simulink model "deliverable_1_simulink"  (R2026a)
settings: Solver=ode4  StopTime=20  FixedStep=0.01
settings Model: Creator=20253802  LastModifiedBy=20253802

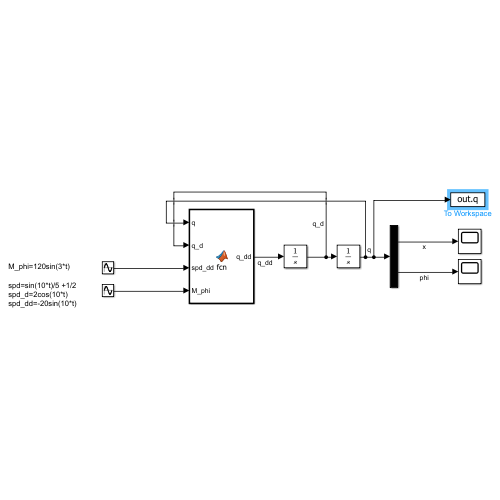
[thumbnail: Simulink's stored preview of the top-level diagram]
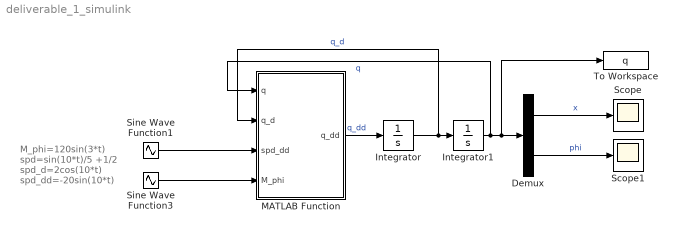
== system deliverable_1_simulink ==
  note: M_phi=120sin(3*t)
      |
      | spd=sin(10*t)/5 +1/2
      | spd_d=2cos(10*t)
      | spd_dd=-20sin(10*t)
  Demux : Demux  Outputs=2
  Integrator : Integrator  InitialCondition=[0 ; 0]
  Integrator1 : Integrator  InitialCondition=[0.1; -pi/4]
  MATLAB Function : MATLAB Function  TreatAsAtomicUnit=on
  Scope : Scope
      settings: ActiveDisplayYMinimum=0.2439492742252623  ActiveDisplayYMaximum=0.82436014260747192
  Scope1 : Scope
      settings: ActiveDisplayYMinimum=-3.2356158180174166  ActiveDisplayYMaximum=0.652208178898841
  Sine Wave Function1 : Sin  Amplitude=-20  Frequency=10  SampleTime=0
  Sine Wave Function3 : Sin  Amplitude=120  Frequency=3  SampleTime=0
  To Workspace : ToWorkspace  VariableName=q  SaveFormat=Timeseries  SampleTime=-1
  wires:
  MATLAB Function/1(q_dd) -> Integrator/1  "q_dd"
  Integrator/1 -> MATLAB Function/2(q_d), Integrator1/1  "q_d"
  Integrator1/1 -> To Workspace/1, Demux/1, MATLAB Function/1(q)  "q"
  Sine Wave Function1/1 -> MATLAB Function/3(spd_dd)
  Sine Wave Function3/1 -> MATLAB Function/4(M_phi)
  Demux/1 -> Scope/1  "x"
  Demux/2 -> Scope1/1  "phi"

== matlab function deliverable_1_simulink/MATLAB Function ==
  data: q input; q_dd output; q_d input; spd_dd input; M_phi input
function q_dd = fcn(q,q_d,spd_dd,M_phi)
%% System Parameters

% Gravitational acceleration
g = 9.81;               % [m/s^2]

% Geometry
L23 = 0.05;             % Distance between points 2 and 3 [m]

% Masses
mc = 2.0;               % Mass of carriage [kg]
mh = 0.7;               % Mass of milling head [kg]

% Inertia
Jh2 = 1.2;              % Rotational inertia of milling head about point 2 [kg*m^2]

% PD controller (x-direction)
kPD = 380;              % Proportional gain [N/m]
xPD_ref = 0.5;          % Reference position [m]
dPD = 10;               % Derivative gain [N*s/m]

% Translational spring-damper (between points 1 and 2)
dx = 0.5;               % Damping coefficient [N*s/m]

% Rotational spring-damper
kphi = 100;             % Rotational stiffness [N*m/rad]

% For problems except D5.f and D6
dphi = 2;               % Rotational damping [N*m*s/rad]

% Reference angles
phi_ref = -0.5*pi;      % Reference angle of band brake [rad]
phi_h3 = (2/3)*pi;      % Relative angle of milling head [rad]



%Generalised coordinates

x     = q(1);
phi   = q(2);
x_d   = q_d(1);
phi_d = q_d(2);
phi3  = phi-phi_h3;

%Calculate M and F

M = [mc+mh,              -mh*L23*sin(phi3);
    -mh*L23*sin(phi3),   Jh2];

F = [
    mh*L23*cos(phi3)*phi_d^2 - kPD*(x - xPD_ref) - (dx + dPD)*x_d ;

    M_phi - mh*L23*cos(phi3)*spd_dd - mh*g*L23*cos(phi3) - kphi*(phi - phi_ref) - dphi*phi_d
    ];


%Solve M q_dd = F 

q_dd = M\F;
